simulink model "SMC_EKF_simulation"  (R2025a)
settings: Solver=ode4  StartTime=0.0  StopTime=200  FixedStep=0.001  RelTol=1e-3
undefined symbols (not defined in the file or in its folder): p
libraries: sharedTrackingLibrary x1
settings Model: Creator=Giammo  LastModifiedBy=Giammo
settings DebuggingCC: MergeDetectMultiDrivingBlocksExec=none
settings ModelReferenceCC: PropagateSignalLabelsOutOfModel=off

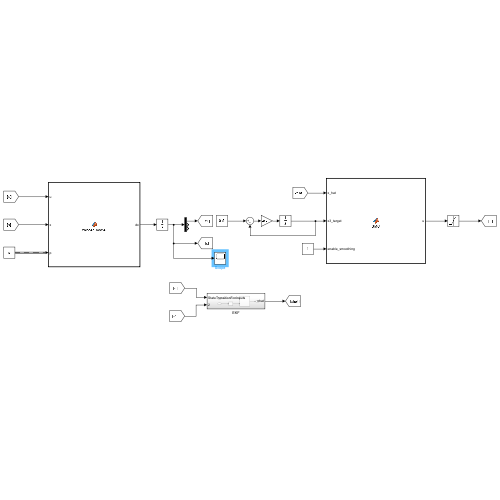
[thumbnail: Simulink's stored preview of the top-level diagram]
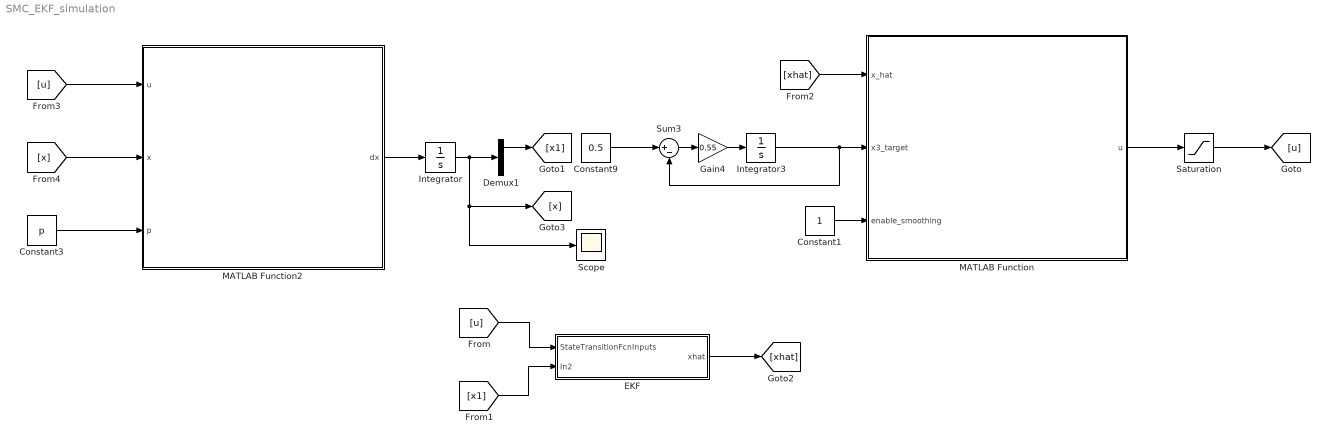
== system SMC_EKF_simulation ==
  Constant1 : Constant
  Constant3 : Constant  Value=p  OutDataTypeStr=Bus: slBus1
  Constant9 : Constant  Value=0.5
  Demux1 : Demux  Outputs=3
  EKF : Subsystem
  Gain4 : Gain  Gain=0.55
  Integrator : Integrator  InitialCondition=[0.1;0.1;0.1]
  Integrator3 : Integrator  InitialCondition=0.5
  MATLAB Function : MATLAB Function  TreatAsAtomicUnit=on
  MATLAB Function2 : MATLAB Function  TreatAsAtomicUnit=on
  Saturation : Saturate  UpperLimit=1  LowerLimit=0
  Scope : Scope
      settings: ActiveDisplayYMinimum=-0.12499999999998841  ActiveDisplayYMaximum=1.1249999999998959
  Sum3 : Sum  Inputs=|+-
  wires:
  Constant3/1 -> MATLAB Function2/3(p)
  MATLAB Function2/1(dx) -> Integrator/1
  Constant1/1 -> MATLAB Function/3(enable_smoothing)
  MATLAB Function/1(u) -> Saturation/1
  [u] -> MATLAB Function2/1(u)
  Demux1/1 -> [x1]
  Saturation/1 -> [u]
  Constant9/1 -> Sum3/1
  Sum3/1 -> Gain4/1
  Gain4/1 -> Integrator3/1
  Integrator3/1 -> MATLAB Function/2(x3_target), Sum3/2
  Integrator/1 -> Scope/1, [x], Demux1/1
  [x] -> MATLAB Function2/2(x)
  [u] -> EKF/1(StateTransitionFcnInputs)
  [x1] -> EKF/2(In2)
  EKF/1(xhat) -> [xhat]
  [xhat] -> MATLAB Function/1(x_hat)

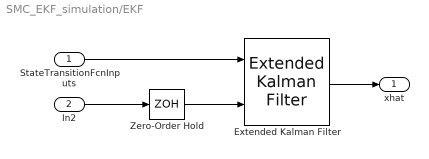
== system SMC_EKF_simulation/EKF ==
  StateTransitionFcnInputs : Inport
  In2 : Inport  Port=2
  Extended Kalman Filter : sharedTrackingLibrary/Extended Kalman Filter  StateTransitionFcn=TDCM_StateTransition  HasStateTransitionJacobianFcn=on  StateTransitionJacobianFcn=TDCM_Jacobian  HasAdditiveProcessNoise=Additive  ProcessNoise=diag([1e-6, 1e-1, 1e-6])  HasTimeVaryingProcessNoise=off  HasStateTransitionFcnExtraArgument=1  InitialState=[0.3;0.5;0.6]  InitialStateCovariance=[1e-9;1e-9;1e-9]  MeasurementFcn1=TDCM_OutputMapping  HasMeasurementJacobianFcn1=on  MeasurementJacobianFcn1=TDCM_MeasJacobian  HasMeasurementEnablePort1=off  HasAdditiveMeasurementNoise1=Additive  MeasurementNoise1=1e-6  HasTimeVaryingMeasurementNoise1=off  HasMeasurementFcnExtraArgument1=0  HasMeasurementWrapping1=off  MeasurementFcn2=myMeasurementFcn  HasMeasurementJacobianFcn2=off  HasMeasurementEnablePort2=off  HasAdditiveMeasurementNoise2=Additive  MeasurementNoise2=1  HasTimeVaryingMeasurementNoise2=off  HasMeasurementFcnExtraArgument2=0  HasMeasurementWrapping2=off  MeasurementFcn3=myMeasurementFcn  HasMeasurementJacobianFcn3=off  HasMeasurementEnablePort3=off  HasAdditiveMeasurementNoise3=Additive  MeasurementNoise3=1  HasTimeVaryingMeasurementNoise3=off  HasMeasurementFcnExtraArgument3=0  HasMeasurementWrapping3=off  MeasurementFcn4=myMeasurementFcn  HasMeasurementJacobianFcn4=off  HasMeasurementEnablePort4=off  HasAdditiveMeasurementNoise4=Additive  MeasurementNoise4=1  HasTimeVaryingMeasurementNoise4=off  HasMeasurementFcnExtraArgument4=0  HasMeasurementWrapping4=off  MeasurementFcn5=myMeasurementFcn  HasMeasurementJacobianFcn5=off  HasMeasurementEnablePort5=off  HasAdditiveMeasurementNoise5=Additive  MeasurementNoise5=1  HasTimeVaryingMeasurementNoise5=off  HasMeasurementFcnExtraArgument5=0  HasMeasurementWrapping5=off  EnableMultirate=off  StateTransitionFcnSampleTime=1  MeasurementFcn1SampleTime=1  MeasurementFcn2SampleTime=1  MeasurementFcn3SampleTime=1  MeasurementFcn4SampleTime=1  MeasurementFcn5SampleTime=1  UseCurrentEstimator=on  OutputStateCovariance=off  DataType=double  SampleTime=0.001  NumberOfMeasurements=1
  Zero-Order Hold : ZeroOrderHold  SampleTime=0.001
  xhat : Outport
  wires:
  Zero-Order Hold/1 -> Extended Kalman Filter/2
  In2/1 -> Zero-Order Hold/1
  StateTransitionFcnInputs/1 -> Extended Kalman Filter/1
  Extended Kalman Filter/1 -> xhat/1

== matlab function SMC_EKF_simulation/MATLAB Function ==
  settings: updateMethod=DISCRETE  sampleTime=0.001
  data: x_hat input size=[3 1]; u output; x3_target input; enable_smoothing input
function u = SMC(x_hat, x3_target, enable_smoothing)
    % Compute sliding mode control from the EKF state estimate.
    R3 = 4.5; D3 = 0.5; A31 = 0.2; k3 = 1.0;
    
    x1_est = x_hat(1);
    x3_est = x_hat(3); 
    
    lambda = 2.0; 
    sigma = lambda * (x3_est - x3_target);
    error = x3_est - x3_target;

    % Evaluate the nominal resting-cell drift using the estimated states.
    f3_hat = (R3 * x1_est * x3_est) / (x1_est + k3) - ...
             A31 * x1_est * x3_est - D3 * x3_est;
    
    K = 10.0; 
    u_eq = -f3_hat; 
    
    % Select sign switching or a smooth tanh approximation.
    if enable_smoothing == 0
        u_sw = -(K / lambda) * sign(sigma);
    else
        phi = 1; 
        u_sw = -(K / lambda) * tanh(sigma / phi);
    end
    
    u_ideal = u_eq + u_sw;
    u = u_ideal;
end

== matlab function SMC_EKF_simulation/MATLAB Function2 ==
  data: u input; dx output; x input; p input
function dx = cancer_model(u, x, p)
    % Continuous-time dynamics: states are tumor, hunting cells and resting cells; u acts on x3.

    x1 = x(1);
    x2 = x(2);
    x3 = x(3);
    
    A12 = p.A12;
    A13 = p.A13;
    R2  = p.R2;
    A21 = p.A21;
    R3  = p.R3;
    k3  = p.k3;
    A31 = p.A31;
    D3  = p.D3;

    dx = zeros(3,1);

    
    dx(1) = x1*(1 - x1) - A12*x1*x2 - A13*x1*x3;

    dx(2) = R2*x2*(1 - x2) - A21*x1*x2;

    recruitment = (R3 * x1 * x3) / (x1 + k3);
    dx(3) = recruitment - A31*x1*x3 - D3*x3 + u;

end
